simulink model "furuta_block_model_fixed_ppo_swingup"  (R2026b)
settings: Solver=ode14x  StopTime=25  FixedStep=driveElectrical.sampleTime
InitFcn:
  | validate_furuta_fixed_test(bdroot);
model workspace (MAT data in the model file):
  calibration = [73.65 -1 4058.5 1]
  controlPeriod = 0.01
  drive = [-1 1.5 1.5 inf]
  driveElectrical : object (value not decoded)
  failureReplayEnabled = 0
  failureReplaySlowdown = 10
  failureReplaySource = 'C:\Capstone1\matlab_furuta\results\ppo_rmd_candidate_tpa79dc374_f9fe_4d66_a12a_2e210f4a8415\ppo_start_-20_+20_armrate_20_current_1.5_time_10_armlimit_Inf.mat'
  failureReplayStartDeg = 20
  failureReplayState = [0 0.1 0.2 0.3 0.4 0.5 0.6 0.7 0.8 0.9 1 1.1 ... (205 elements, 41x5)]
  furutaPPOAgent : rl.agent.rlPPOAgent (value not decoded)
  furutaSACAgent : rl.agent.rlSACAgent (value not decoded)
  furutaToolboxMpc : object (value not decoded)
  initialState = [0; 3.14159265359; 0; 0]
  integrationStep = 0.002
  limits = [inf 3.3 15 20]
  lqrGain = [-1.90684760658 -25.0276005412 -1.03983138576 -2.50199272238]
  maxTorque = 3.15
  milVelocityLimits = [15 25]
  pidGains = [25.0276005412 5.00398544475 1.90684760658 2.07966277151 0.001]
  plantCoefficients = [0.05 0.00016078 0.00016134 0.00013805 0.016934 0.0001 1e-05 0.63]
  rlRewardLevel = 2
  rmd : object (value not decoded)
  rmdCommandDelaySamples = 1
  scenarioStimulus = [0  0  0  0; 20  0  0  0]
  swingLqrThresholds = [0.226892802759 0.2 0.523598775598]
  usePolicyCallback = 0
  useRmd = 1
  velocityFilterTau = 0.03
values from neighbouring files (symbols this model uses):
  C = [B A*B A^2*B A^3*B]    [build_furuta_rmd.m]
  N = 20    [build_furuta_rl.m]    (also in design_classical.m)
  s = load(matFile,'ds')    [analyze_pi_current_run.m]    (also in analyze_pi_speed_run.m; build_furuta_rl.m = sin(x(2));"; build_furuta_simulink.m = s(1); design_classical.m = furuta_scenarios)
  source = [step '/1']    [add_furuta_plant_blocks.m]    (also in build_furuta_pi.m = get_param(line,'SrcPortHandle'); build_furuta_pi_hardware.m = 'Drive interlocks/3'; compare_furuta_actuators.m = get_param([harness '/Requested torque'],'PortHandles'))
  Z = expm([A B; zeros(1,5)]*p.Ts)    [furuta_linearize.m]
symbols that are objects in the model workspace (value not decoded): driveElectrical, rmd
undefined symbols (not defined in the file or in its folder): lmpcF, lmpcH, poleGain, sgn, X, Y
libraries: sm_lib x36, raspberrypiCommlib x9, nesl_utility x8, fl_lib x7, rllib x2, mpclib x1, slpidlib x1, ee_lib x1
(part 3 of 4)

== system furuta_block_model_fixed_ppo_swingup/01 MIL - Controller and Plant/03 Controllers/PID ==
  mode : Inport
  x : Inport  Port=2
  Arm reference log : ToWorkspace  VariableName=swingPIDArmHome  SaveFormat=Timeseries  SampleTime=-1
  Capture arm reference : MATLAB Function  TreatAsAtomicUnit=on
  Capture thresholds : Constant  Value=swingLqrThresholds
  Control period : Constant  Value=controlPeriod
  Energy parameters : Constant  Value=plantCoefficients
  PID Controller : slpidlib/PID Controller  Controller=PID  Form=Parallel  TimeDomain=Continuous-time  UseExternalTs=off  SampleTime=-1  IntegratorMethod=Forward Euler  FilterMethod=Forward Euler  ControllerParametersSource=internal  P=1  I=1  UseKiTs=off  D=0  UseExternalDerivativeSource=off  N=100  UseFilter=on  TunerSelectOption=Transfer Function Based (PID Tuner App)  InitialConditionSource=internal  InitialConditionForIntegrator=0  InitialConditionForFilter=0  DifferentiatorICPrevScaledInput=0  ExternalReset=none  TrackingMode=off  Kt=1  LimitOutput=off  SatLimitsSource=internal  UpperSaturationLimit=inf  LowerSaturationLimit=-inf  LinearizeAsGain=on  AntiWindupMode=none  Kb=1  LimitIntegrator=off  UpperIntegratorSaturationLimit=inf  LowerIntegratorSaturationLimit=-inf  POutMin=[]  POutMax=[]  IOutMin=[]  IOutMax=[]  DOutMin=[]  DOutMax=[]  NOutMin=[]  NOutMax=[]  SumOutMin=[]  SumOutMax=[]  SaturationOutMin=[]  SaturationOutMax=[]  PParamMin=[]  PParamMax=[]  IParamMin=[]  IParamMax=[]  DParamMin=[]  DParamMax=[]  NParamMin=[]  NParamMax=[]  KbParamMin=[]  KbParamMax=[]  KtParamMin=[]  KtParamMax=[]  KbOutMin=[]  KbOutMax=[]  KtOutMin=[]  KtOutMax=[]  IntegratorOutMin=[]  IntegratorOutMax=[]  FilterOutMin=[]  FilterOutMax=[]  SumI1OutMin=[]  SumI1OutMax=[]  SumI2OutMin=[]  SumI2OutMax=[]  SumI3OutMin=[]  SumI3OutMax=[]  SumI4OutMin=[]  SumI4OutMax=[]  SumDOutMin=[]  SumDOutMax=[]  DifferentiatorOutMin=[]  DifferentiatorOutMax=[]  FilterDiffOutCoefMin=[]  FilterDiffOutCoefMax=[]  ReciprocalOutMin=[]  ReciprocalOutMax=[]  SumDenOutMin=[]  SumDenOutMax=[]  SumNumOutMin=[]  SumNumOutMax=[]  DivideOutMin=[]  DivideOutMax=[]  UdiffTsProdOutMin=[]  UdiffTsProdOutMax=[]  NTsProdOutMin=[]  NTsProdOutMax=[]  UintegralTsProdOutMin=[]  UintegralTsProdOutMax=[]  UngainTsProdOutMin=[]  UngainTsProdOutMax=[]  ClampingZeroOutDataTypeStr=Inherit: Inherit via back propagation  ClampingZeroOutMin=[]  ClampingZeroOutMax=[]  FilterDenConstantOutDataTypeStr=Inherit: Inherit via back propagation  FilterDenConstantOutMin=[]  FilterDenConstantOutMax=[]  PCopyOutDataTypeStr=Inherit: Inherit via back propagation  PCopyOutMin=[]  PCopyOutMax=[]  NCopyOutDataTypeStr=Inherit: Inherit via back propagation  NCopyOutMin=[]  NCopyOutMax=[]  IntegratorContinuousStateAttributes=''  IntegratorStateMustResolveToSignalObject=off  IntegratorRTWStateStorageClass=Auto  FilterContinuousStateAttributes=''  FilterStateMustResolveToSignalObject=off  FilterRTWStateStorageClass=Auto  ParallelPVariant=InternalParameters  IdealPVariant=Disabled  IVariant=InternalParameters  DVariant=InternalParameters  IntegratorVariant=Continuous  SatVariant=Disabled  AWVariant=Passthrough  PCopyVariant=Disabled  TRVariant=Disabled  FdbkBlocksVariant=Forward  IdealPFdbkVariant=Disabled  SatFdbkVariant=Disabled  DerivativeFilterVariant=ContFilter  NVariant=InternalParameters  NCopyVariant=Disabled  FilterICVariant=InternalICsFilter  IntegratorICVariant=InternalICs  ExternalResetVariant=Disabled  TRSumVariant=Passthrough  SumFdbkVariant=Disabled  SumVariant=Sum_PID  TsampFilterVariant=InternalTs  TsampNgainVariant=Passthrough  TsampIntegralVariant=Disabled_SignalSpec  ExternalSaturationOutDataTypeStr=Inherit: Same as second input  DerivativeSourceVariant=ErrorSignal  PreIntVariant=InternalPreInt
  PID active log : ToWorkspace  VariableName=swingPIDActive  SaveFormat=Timeseries  SampleTime=-1
  PID gains : Constant  Value=pidGains
  PID with anti windup : MATLAB Function  TreatAsAtomicUnit=on
  Swing-up to PID : MATLAB Function  TreatAsAtomicUnit=on
  u : Outport
  wires:
  PID gains/1 -> PID with anti windup/2(g)
  Control period/1 -> PID with anti windup/3(dt)
  x/1 -> Swing-up to PID/1(x), Capture arm reference/1(x)
  mode/1 -> Swing-up to PID/3(mode), Capture arm reference/2(mode)
  PID with anti windup/1(u) -> Swing-up to PID/2(balance)
  Capture thresholds/1 -> Swing-up to PID/4(thresholds), Capture arm reference/3(thresholds)
  Energy parameters/1 -> Swing-up to PID/5(p)
  Swing-up to PID/1(u) -> u/1
  Swing-up to PID/2(balancing) -> PID active log/1
  Capture arm reference/1(relative) -> PID with anti windup/1(x)
  Capture arm reference/2(gatedMode) -> PID with anti windup/4(mode)
  Capture arm reference/3(home) -> Arm reference log/1

== system furuta_block_model_fixed_ppo_swingup/01 MIL - Controller and Plant/03 Controllers/PPO ==
  Controller mode : Inport
  Measured state : Inport  Port=2
  Previous RL action : UnitDelay  SampleTime=controlPeriod
  RL Agent : rllib/RL Agent  Agent=furutaPPOAgent  ExternalActionAsInput=off  ProvideLastAction=off  ProvideCumRwd=off  TreatAsDirectFeedthrough=on  UseStrictObservationDataTypes=off
  RL action limit : Saturate  UpperLimit=1  LowerLimit=-1
  RL observation reward termination : MATLAB Function  TreatAsAtomicUnit=on
  Reward level : Constant  Value=rlRewardLevel
  Out1 : Outport
  wires:
  Controller mode/1 -> RL observation reward termination/1(x)
  RL observation reward termination/3(done) -> RL Agent/3
  RL Agent/1 -> RL action limit/1
  RL observation reward termination/2(reward) -> RL Agent/2
  Previous RL action/1 -> RL observation reward termination/2(lastAction)
  RL action limit/1 -> Out1/1, Previous RL action/1
  RL observation reward termination/1(obs) -> RL Agent/1
  Reward level/1 -> RL observation reward termination/3(level)
  Measured state/1 -> RL observation reward termination/4(mode)

== system furuta_block_model_fixed_ppo_swingup/01 MIL - Controller and Plant/03 Controllers/Pendulum and arm PD ==
  mode : Inport
  x : Inport  Port=2
  Control period : Constant  Value=controlPeriod
  Pendulum and arm PD : Gain  Gain=[.50 8.0 .29 .58]  Multiplication=Matrix(K*u) (u vector)
  u : Outport
  wires:
  Control period/1 -> ?
  mode/1 -> ?
  Pendulum and arm PD/1 -> u/1
  x/1 -> Pendulum and arm PD/1

== system furuta_block_model_fixed_ppo_swingup/01 MIL - Controller and Plant/03 Controllers/Pole placement ==
  mode : Inport
  x : Inport  Port=2
  Control period : Constant  Value=controlPeriod
  Pole placement : Gain  Gain=-poleGain  Multiplication=Matrix(K*u) (u vector)
  u : Outport
  wires:
  Control period/1 -> ?
  mode/1 -> ?
  Pole placement/1 -> u/1
  x/1 -> Pole placement/1

== system furuta_block_model_fixed_ppo_swingup/01 MIL - Controller and Plant/03 Controllers/SAC ==
  x : Inport
  mode : Inport  Port=2
  Previous RL action : UnitDelay  SampleTime=controlPeriod
  RL Agent : rllib/RL Agent  Agent=furutaSACAgent  ExternalActionAsInput=off  ProvideLastAction=off  ProvideCumRwd=off  TreatAsDirectFeedthrough=on  UseStrictObservationDataTypes=off
  RL action limit : Saturate  UpperLimit=1  LowerLimit=-1
  RL observation reward termination : MATLAB Function  TreatAsAtomicUnit=on
  Reward level : Constant  Value=rlRewardLevel
  Out1 : Outport
  wires:
  x/1 -> RL observation reward termination/1(x)
  RL observation reward termination/3(done) -> RL Agent/3
  RL Agent/1 -> RL action limit/1
  RL observation reward termination/2(reward) -> RL Agent/2
  Previous RL action/1 -> RL observation reward termination/2(lastAction)
  RL action limit/1 -> Out1/1, Previous RL action/1
  RL observation reward termination/1(obs) -> RL Agent/1
  Reward level/1 -> RL observation reward termination/3(level)
  mode/1 -> RL observation reward termination/4(mode)

== system furuta_block_model_fixed_ppo_swingup/01 MIL - Controller and Plant/04 Actuator/RMD X6 P20 60 E ==
  Output shaft speed : Inport
  Requested torque : Inport  Port=2
  01 RMD Driver : Subsystem
  02 RMD Motor : Subsystem
  Output torque : Outport
  wires:
  Requested torque/1 -> 01 RMD Driver/2(Requested torque)
  Output shaft speed/1 -> 02 RMD Motor/1(Output shaft speed)
  02 RMD Motor/1(output) -> 01 RMD Driver/1(output)
  02 RMD Motor/2(input0) -> 01 RMD Driver/3(input0)
  02 RMD Motor/3(Output torque) -> Output torque/1
  connections:
  01 RMD Driver/RConn1 -- 02 RMD Motor/LConn1
  02 RMD Motor/RConn1 -- 01 RMD Driver/LConn1

== system furuta_block_model_fixed_ppo_swingup/01 MIL - Controller and Plant/05 Furuta plant/RK4 Furuta plant ==
  state : Inport
  total torque : Inport  Port=2
  Substep 1 : Subsystem
  Substep 2 : Subsystem
  Substep 3 : Subsystem
  Substep 4 : Subsystem
  Substep 5 : Subsystem
  next state : Outport
  wires:
  state/1 -> Substep 1/1(x)
  total torque/1 -> Substep 4/2(tau), Substep 5/2(tau), Substep 3/2(tau), Substep 2/2(tau), Substep 1/2(tau)
  Substep 1/1(x next) -> Substep 2/1(x)
  Substep 2/1(x next) -> Substep 3/1(x)
  Substep 3/1(x next) -> Substep 4/1(x)
  Substep 4/1(x next) -> Substep 5/1(x)
  Substep 5/1(x next) -> next state/1

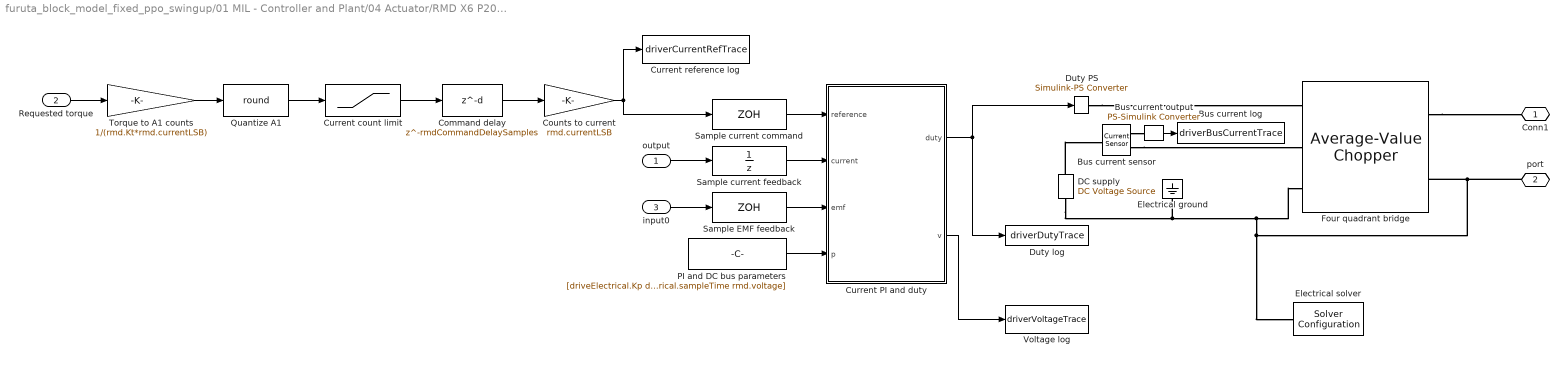
== system furuta_block_model_fixed_ppo_swingup/01 MIL - Controller and Plant/04 Actuator/RMD X6 P20 60 E/01 RMD Driver ==
  output : Inport
  Requested torque : Inport  Port=2
  input0 : Inport  Port=3
  Bus current log : ToWorkspace  VariableName=driverBusCurrentTrace  SaveFormat=Timeseries  SampleTime=-1
  Bus current output : nesl_utility/PS-Simulink Converter  PhysicalDomain=network_engine_domain  SubClassName=ps_output  LeftPortType=input  RightPortType=output  PseudoPeriodic=off  Frequencies=[]  VectorFormat=inherit  Unit=A  AffineConversion=off
  Bus current sensor : fl_lib/Electrical/Electrical Sensors/Current Sensor
  Command delay : Delay  DelayLength=rmdCommandDelaySamples  SampleTime=controlPeriod
  Counts to current : Gain  Gain=rmd.currentLSB
  Current PI and duty : MATLAB Function  TreatAsAtomicUnit=on
  Current count limit : Saturate  UpperLimit=floor(min([maxTorque/rmd.Kt rmd.ratedTorque/rmd.Kt rmd.ratedCurrent])/rmd.currentLSB)  LowerLimit=-(floor(min([maxTorque/rmd.Kt rmd.ratedTorque/rmd.Kt rmd.ratedCurrent])/rmd.currentLSB))
  Current reference log : ToWorkspace  VariableName=driverCurrentRefTrace  SaveFormat=Timeseries  SampleTime=-1
  DC supply : fl_lib/Electrical/Electrical Sources/DC Voltage Source  v0=rmd.voltage V
  Duty PS : nesl_utility/Simulink-PS Converter  PhysicalDomain=network_engine_domain  SubClassName=ps_input  LeftPortType=input  RightPortType=output  PseudoPeriodic=off  Frequencies=[]  NoiseDistribution=none  NoiseParameters=[]  Unit=1  AffineConversion=off  FilteringAndDerivatives=zero  SimscapeFilterOrder=1  InputFilterTimeConstant=0.001  UdotUserProvided=0
  Duty log : ToWorkspace  VariableName=driverDutyTrace  SaveFormat=Timeseries  SampleTime=-1
  Electrical ground : fl_lib/Electrical/Electrical Elements/Electrical Reference
  Electrical solver : nesl_utility/Solver Configuration  PhysicalDomain=network_engine_domain  SubClassName=solver  LeftPortType=input  RightPortType=generic  Tones=[]  Harmonics=[]  SimulateNoise=off  Profile=off  UseLocalSampling=off  EnableSwitchedLinearOptims=on  FrequencyDomain=off  UseCCode=off  RelTol=0.001  AbsTol=0.001  MinStep=1e-09  ToWorkspace=off  RevertToSquareIcSolve=off  NumHomotopyIterations=100  PhasorMode=off  PhasorModeNumHarmonics=1  ConsistencySolver=NEWTON_XTOL_AFTER_FTOL  CanonicalOrdering=CANONICAL  OptimizeIntermediates=OPTIMIZED  MulticoreSolverChoice=BACKWARD_EULER  IndexReductionMethod=DerivativeReplacement  DoDC=off  ResidualTolerance=1e-09  ConsistencyTolSource=GLOBAL  ConsistencyAbsTol=0.001  ConsistencyRelTol=0.001  ConsistencyTolFactor=0.001  UseLocalSolver=off  LocalSolverChoice=NE_BACKWARD_EULER_ADVANCER  ResolveIndetEquations=on  FunctionEvalNumThread=1  LocalSolverSampleTime=0.001  DoFixedCost=off  MaxNonlinIter=3  MaxModeIter=2  ComputeImpulses=off  ImpulseIterations=2  LinearAlgebra=auto  LinearAlgebraNumThread=0  EquationFormulation=NE_TIME_EF  DelaysMemoryBudget=1024  AutomaticFiltering=on  FilteringTimeConstant=0.001  PartitionStorageMethod=AS_NEEDED  PartitionMemoryBudget=1024  PartitionMethod=BALANCED  MultibodyUseLocalSolver=off  MultibodyLocalSolverChoice=ODE1  MultibodyLocalSolverSampleTime=0.001
  Four quadrant bridge : ee_lib/Semiconductors & Converters/Converters/Average-Value Chopper  chopper_type=ee.enum.converters.averageChopperType.classE  efficiency_option=ee.enum.converters.efficiencyOption.constant  efficiency_fixed=100  i_vec=[0, 2, 5] A  efficiency_vec=[90, 95, 98]
  PI and DC bus parameters : Constant  Value=[driveElectrical.Kp driveElectrical.Ki driveElectrical.sampleTime rmd.voltage]
  Quantize A1 : Rounding  Operator=round
  Sample EMF feedback : ZeroOrderHold  SampleTime=driveElectrical.sampleTime
  Sample current command : ZeroOrderHold  SampleTime=driveElectrical.sampleTime
  Sample current feedback : UnitDelay  SampleTime=driveElectrical.sampleTime
  Torque to A1 counts : Gain  Gain=1/(rmd.Kt*rmd.currentLSB)
  Voltage log : ToWorkspace  VariableName=driverVoltageTrace  SaveFormat=Timeseries  SampleTime=-1
  Conn1 : PMIOPort  Side=Right
  port : PMIOPort  Port=2  Side=Left
  wires:
  Torque to A1 counts/1 -> Quantize A1/1
  Command delay/1 -> Counts to current/1
  Bus current output/1 -> Bus current log/1
  Sample current command/1 -> Current PI and duty/1(reference)
  Counts to current/1 -> Current reference log/1, Sample current command/1
  Current count limit/1 -> Command delay/1
  Quantize A1/1 -> Current count limit/1
  Current PI and duty/1(duty) -> Duty PS/1, Duty log/1
  Sample current feedback/1 -> Current PI and duty/2(current)
  input0/1 -> Sample EMF feedback/1
  Current PI and duty/2(v) -> Voltage log/1
  Sample EMF feedback/1 -> Current PI and duty/3(emf)
  PI and DC bus parameters/1 -> Current PI and duty/4(p)
  output/1 -> Sample current feedback/1
  Requested torque/1 -> Torque to A1 counts/1
  connections:
  Bus current sensor/RConn1 -- Bus current output/LConn1
  port/RConn1 -- Four quadrant bridge/RConn2 -- Electrical solver/RConn1 -- Four quadrant bridge/LConn3 -- DC supply/RConn1 -- Electrical ground/LConn1
  Duty PS/RConn1 -- Four quadrant bridge/LConn1
  DC supply/LConn1 -- Bus current sensor/LConn1
  Bus current sensor/RConn2 -- Four quadrant bridge/LConn2
  Four quadrant bridge/RConn1 -- Conn1/RConn1

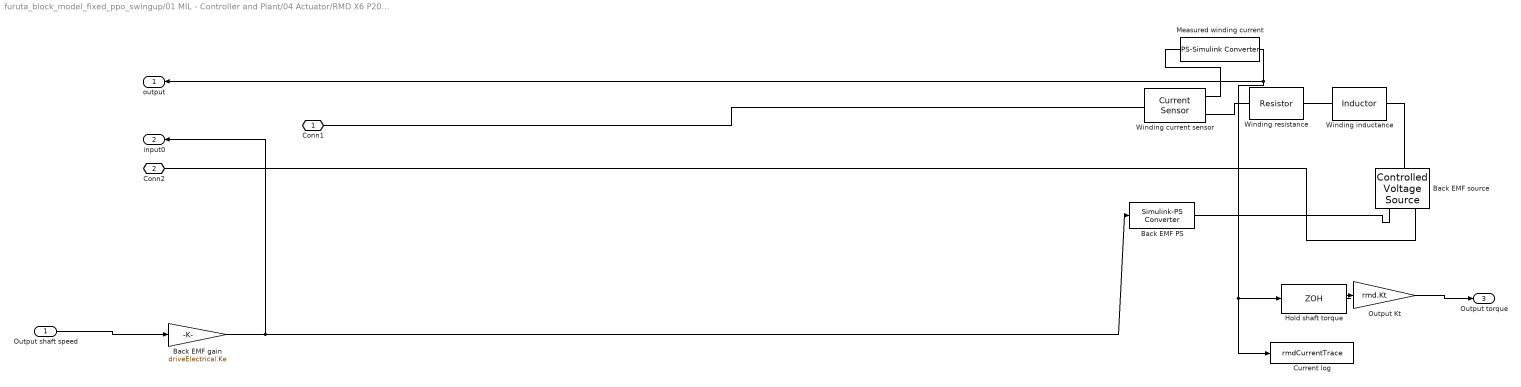
== system furuta_block_model_fixed_ppo_swingup/01 MIL - Controller and Plant/04 Actuator/RMD X6 P20 60 E/02 RMD Motor ==
  Output shaft speed : Inport
  Back EMF PS : nesl_utility/Simulink-PS Converter  PhysicalDomain=network_engine_domain  SubClassName=ps_input  LeftPortType=input  RightPortType=output  PseudoPeriodic=off  Frequencies=[]  NoiseDistribution=none  NoiseParameters=[]  Unit=V  AffineConversion=off  FilteringAndDerivatives=zero  SimscapeFilterOrder=1  InputFilterTimeConstant=0.001  UdotUserProvided=0
  Back EMF gain : Gain  Gain=driveElectrical.Ke
  Back EMF source : fl_lib/Electrical/Electrical Sources/Controlled Voltage Source
  Current log : ToWorkspace  VariableName=rmdCurrentTrace  SampleTime=-1
  Hold shaft torque : ZeroOrderHold  SampleTime=controlPeriod
  Measured winding current : nesl_utility/PS-Simulink Converter  PhysicalDomain=network_engine_domain  SubClassName=ps_output  LeftPortType=input  RightPortType=output  PseudoPeriodic=off  Frequencies=[]  VectorFormat=inherit  Unit=A  AffineConversion=off
  Output Kt : Gain  Gain=rmd.Kt
  Winding current sensor : fl_lib/Electrical/Electrical Sensors/Current Sensor
  Winding inductance : fl_lib/Electrical/Electrical Elements/Inductor  l=driveElectrical.L H  r=0 Ohm  g=0 1/Ohm  i_specify=off  i_priority=None  i=0 A  i_nominal_specify=off  i_nominal_value=1  i_nominal_unit=A  v_specify=off  v_priority=None  v=0 V  v_nominal_specify=off  v_nominal_value=1  v_nominal_unit=V  i_L_specify=off  i_L_priority=High  i_L=0 A  i_L_nominal_specify=off  i_L_nominal_value=1  i_L_nominal_unit=A
  Winding resistance : fl_lib/Electrical/Electrical Elements/Resistor  R=driveElectrical.R Ohm  i_specify=off  i_priority=None  i=0 A  i_nominal_specify=off  i_nominal_value=1  i_nominal_unit=A  v_specify=off  v_priority=None  v=0 V  v_nominal_specify=off  v_nominal_value=1  v_nominal_unit=V
  Conn1 : PMIOPort  Side=Left
  Conn2 : PMIOPort  Port=2  Side=Right
  output : Outport
  input0 : Outport  Port=2
  Output torque : Outport  Port=3
  wires:
  Measured winding current/1 -> output/1, Hold shaft torque/1, Current log/1
  Output Kt/1 -> Output torque/1
  Hold shaft torque/1 -> Output Kt/1
  Back EMF gain/1 -> Back EMF PS/1, input0/1
  Output shaft speed/1 -> Back EMF gain/1
  connections:
  Back EMF PS/RConn1 -- Back EMF source/RConn1
  Winding current sensor/RConn1 -- Measured winding current/LConn1
  Winding resistance/RConn1 -- Winding inductance/LConn1
  Winding inductance/RConn1 -- Back EMF source/LConn1
  Winding current sensor/RConn2 -- Winding resistance/LConn1
  Conn1/RConn1 -- Winding current sensor/LConn1
  Back EMF source/RConn2 -- Conn2/RConn1

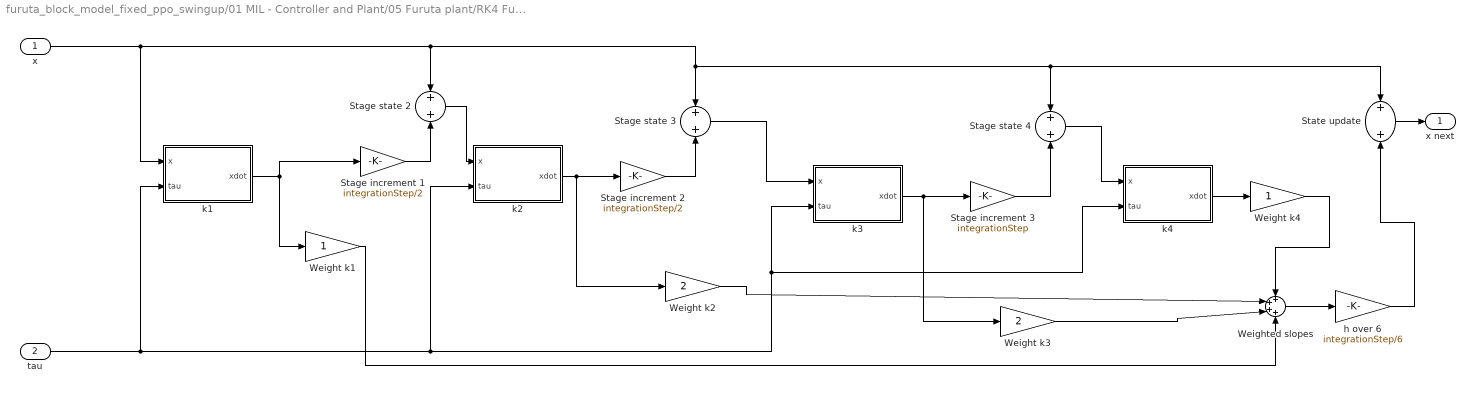
== system furuta_block_model_fixed_ppo_swingup/01 MIL - Controller and Plant/05 Furuta plant/RK4 Furuta plant/Substep 1 ==
  x : Inport
  tau : Inport  Port=2
  Stage increment 1 : Gain  Gain=integrationStep/2
  Stage increment 2 : Gain  Gain=integrationStep/2
  Stage increment 3 : Gain  Gain=integrationStep
  Stage state 2 : Sum
  Stage state 3 : Sum
  Stage state 4 : Sum
  State update : Sum
  Weight k1 : Gain
  Weight k2 : Gain  Gain=2
  Weight k3 : Gain  Gain=2
  Weight k4 : Gain
  Weighted slopes : Sum  Inputs=++++
  h over 6 : Gain  Gain=integrationStep/6
  k1 : Subsystem
  k2 : Subsystem
  k3 : Subsystem
  k4 : Subsystem
  x next : Outport
  wires:
  x/1 -> Stage state 3/1, Stage state 4/1, State update/1, Stage state 2/1, k1/1(x)
  tau/1 -> k4/2(tau), k3/2(tau), k2/2(tau), k1/2(tau)
  k1/1(xdot) -> Stage increment 1/1, Weight k1/1
  Stage increment 1/1 -> Stage state 2/2
  Stage state 2/1 -> k2/1(x)
  k2/1(xdot) -> Stage increment 2/1, Weight k2/1
  Stage increment 2/1 -> Stage state 3/2
  Stage state 3/1 -> k3/1(x)
  k3/1(xdot) -> Weight k3/1, Stage increment 3/1
  Stage increment 3/1 -> Stage state 4/2
  Stage state 4/1 -> k4/1(x)
  k4/1(xdot) -> Weight k4/1
  Weight k1/1 -> Weighted slopes/4
  Weight k2/1 -> Weighted slopes/2
  Weight k3/1 -> Weighted slopes/3
  Weight k4/1 -> Weighted slopes/1
  Weighted slopes/1 -> h over 6/1
  h over 6/1 -> State update/2
  State update/1 -> x next/1

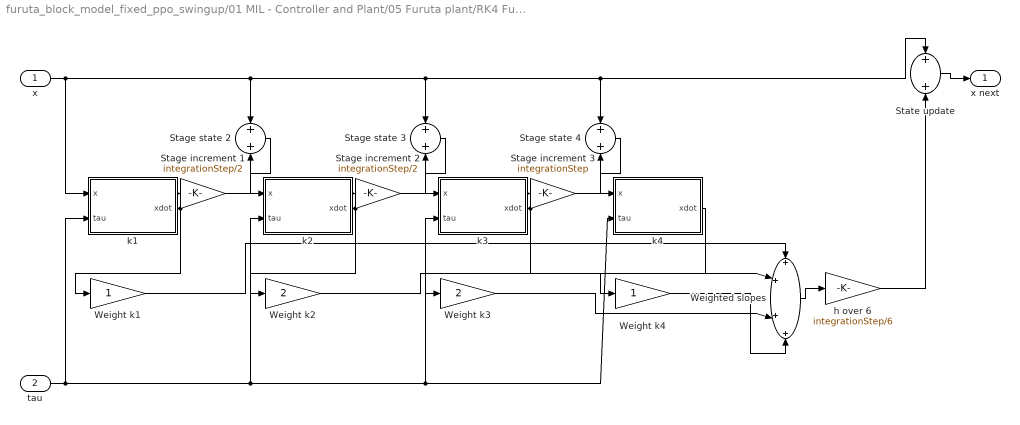
== system furuta_block_model_fixed_ppo_swingup/01 MIL - Controller and Plant/05 Furuta plant/RK4 Furuta plant/Substep 2 ==
  x : Inport
  tau : Inport  Port=2
  Stage increment 1 : Gain  Gain=integrationStep/2
  Stage increment 2 : Gain  Gain=integrationStep/2
  Stage increment 3 : Gain  Gain=integrationStep
  Stage state 2 : Sum
  Stage state 3 : Sum
  Stage state 4 : Sum
  State update : Sum
  Weight k1 : Gain
  Weight k2 : Gain  Gain=2
  Weight k3 : Gain  Gain=2
  Weight k4 : Gain
  Weighted slopes : Sum  Inputs=++++
  h over 6 : Gain  Gain=integrationStep/6
  k1 : Subsystem
  k2 : Subsystem
  k3 : Subsystem
  k4 : Subsystem
  x next : Outport
  wires:
  State update/1 -> x next/1
  h over 6/1 -> State update/2
  Weighted slopes/1 -> h over 6/1
  Weight k4/1 -> Weighted slopes/4
  Weight k3/1 -> Weighted slopes/3
  Weight k2/1 -> Weighted slopes/2
  Weight k1/1 -> Weighted slopes/1
  k4/1(xdot) -> Weight k4/1
  Stage state 4/1 -> k4/1(x)
  Stage increment 3/1 -> Stage state 4/2
  k3/1(xdot) -> Weight k3/1, Stage increment 3/1
  Stage state 3/1 -> k3/1(x)
  Stage increment 2/1 -> Stage state 3/2
  k2/1(xdot) -> Weight k2/1, Stage increment 2/1
  Stage state 2/1 -> k2/1(x)
  Stage increment 1/1 -> Stage state 2/2
  k1/1(xdot) -> Weight k1/1, Stage increment 1/1
  tau/1 -> k4/2(tau), k3/2(tau), k2/2(tau), k1/2(tau)
  x/1 -> State update/1, Stage state 4/1, Stage state 3/1, Stage state 2/1, k1/1(x)

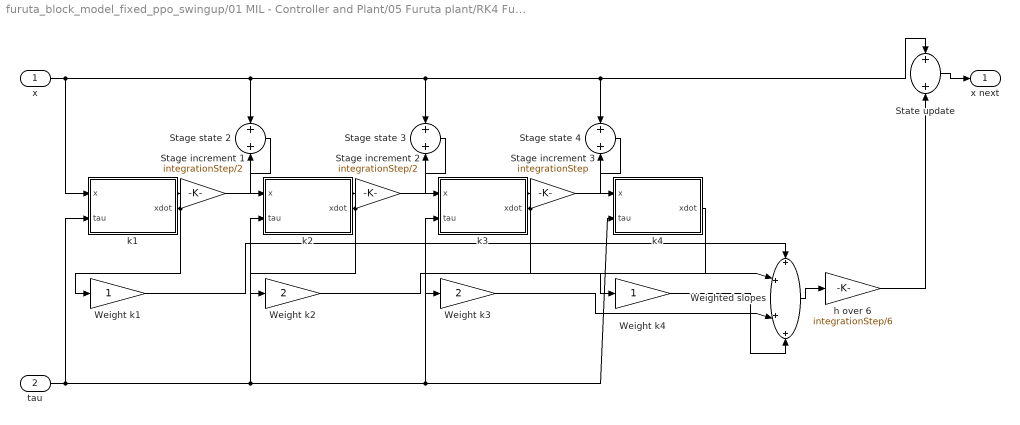
== system furuta_block_model_fixed_ppo_swingup/01 MIL - Controller and Plant/05 Furuta plant/RK4 Furuta plant/Substep 3 ==
  x : Inport
  tau : Inport  Port=2
  Stage increment 1 : Gain  Gain=integrationStep/2
  Stage increment 2 : Gain  Gain=integrationStep/2
  Stage increment 3 : Gain  Gain=integrationStep
  Stage state 2 : Sum
  Stage state 3 : Sum
  Stage state 4 : Sum
  State update : Sum
  Weight k1 : Gain
  Weight k2 : Gain  Gain=2
  Weight k3 : Gain  Gain=2
  Weight k4 : Gain
  Weighted slopes : Sum  Inputs=++++
  h over 6 : Gain  Gain=integrationStep/6
  k1 : Subsystem
  k2 : Subsystem
  k3 : Subsystem
  k4 : Subsystem
  x next : Outport
  wires:
  State update/1 -> x next/1
  h over 6/1 -> State update/2
  Weighted slopes/1 -> h over 6/1
  Weight k4/1 -> Weighted slopes/4
  Weight k3/1 -> Weighted slopes/3
  Weight k2/1 -> Weighted slopes/2
  Weight k1/1 -> Weighted slopes/1
  k4/1(xdot) -> Weight k4/1
  Stage state 4/1 -> k4/1(x)
  Stage increment 3/1 -> Stage state 4/2
  k3/1(xdot) -> Weight k3/1, Stage increment 3/1
  Stage state 3/1 -> k3/1(x)
  Stage increment 2/1 -> Stage state 3/2
  k2/1(xdot) -> Weight k2/1, Stage increment 2/1
  Stage state 2/1 -> k2/1(x)
  Stage increment 1/1 -> Stage state 2/2
  k1/1(xdot) -> Weight k1/1, Stage increment 1/1
  tau/1 -> k4/2(tau), k3/2(tau), k2/2(tau), k1/2(tau)
  x/1 -> State update/1, Stage state 4/1, Stage state 3/1, Stage state 2/1, k1/1(x)

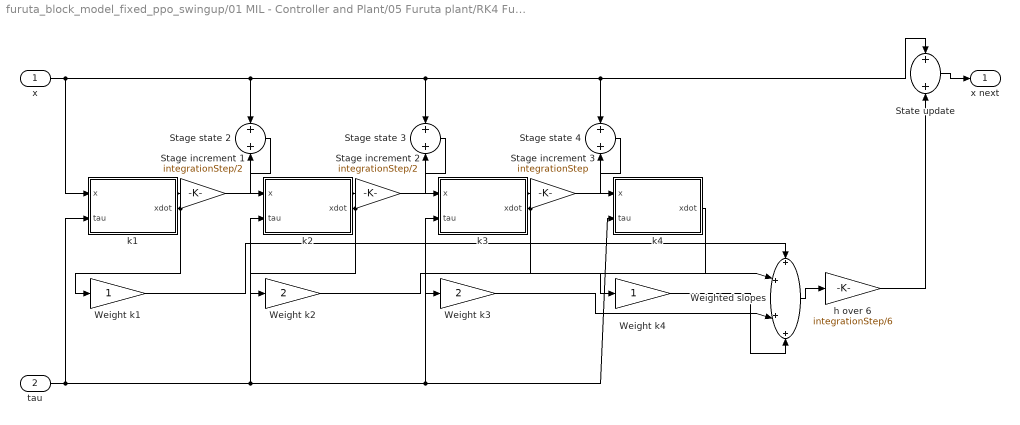
== system furuta_block_model_fixed_ppo_swingup/01 MIL - Controller and Plant/05 Furuta plant/RK4 Furuta plant/Substep 4 ==
  x : Inport
  tau : Inport  Port=2
  Stage increment 1 : Gain  Gain=integrationStep/2
  Stage increment 2 : Gain  Gain=integrationStep/2
  Stage increment 3 : Gain  Gain=integrationStep
  Stage state 2 : Sum
  Stage state 3 : Sum
  Stage state 4 : Sum
  State update : Sum
  Weight k1 : Gain
  Weight k2 : Gain  Gain=2
  Weight k3 : Gain  Gain=2
  Weight k4 : Gain
  Weighted slopes : Sum  Inputs=++++
  h over 6 : Gain  Gain=integrationStep/6
  k1 : Subsystem
  k2 : Subsystem
  k3 : Subsystem
  k4 : Subsystem
  x next : Outport
  wires:
  State update/1 -> x next/1
  h over 6/1 -> State update/2
  Weighted slopes/1 -> h over 6/1
  Weight k4/1 -> Weighted slopes/4
  Weight k3/1 -> Weighted slopes/3
  Weight k2/1 -> Weighted slopes/2
  Weight k1/1 -> Weighted slopes/1
  k4/1(xdot) -> Weight k4/1
  Stage state 4/1 -> k4/1(x)
  Stage increment 3/1 -> Stage state 4/2
  k3/1(xdot) -> Weight k3/1, Stage increment 3/1
  Stage state 3/1 -> k3/1(x)
  Stage increment 2/1 -> Stage state 3/2
  k2/1(xdot) -> Weight k2/1, Stage increment 2/1
  Stage state 2/1 -> k2/1(x)
  Stage increment 1/1 -> Stage state 2/2
  k1/1(xdot) -> Weight k1/1, Stage increment 1/1
  tau/1 -> k4/2(tau), k3/2(tau), k2/2(tau), k1/2(tau)
  x/1 -> State update/1, Stage state 4/1, Stage state 3/1, Stage state 2/1, k1/1(x)

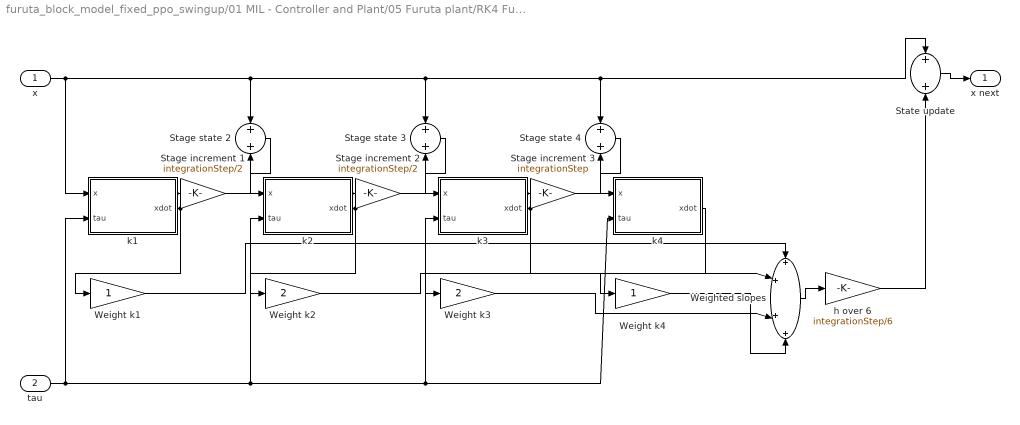
== system furuta_block_model_fixed_ppo_swingup/01 MIL - Controller and Plant/05 Furuta plant/RK4 Furuta plant/Substep 5 ==
  x : Inport
  tau : Inport  Port=2
  Stage increment 1 : Gain  Gain=integrationStep/2
  Stage increment 2 : Gain  Gain=integrationStep/2
  Stage increment 3 : Gain  Gain=integrationStep
  Stage state 2 : Sum
  Stage state 3 : Sum
  Stage state 4 : Sum
  State update : Sum
  Weight k1 : Gain
  Weight k2 : Gain  Gain=2
  Weight k3 : Gain  Gain=2
  Weight k4 : Gain
  Weighted slopes : Sum  Inputs=++++
  h over 6 : Gain  Gain=integrationStep/6
  k1 : Subsystem
  k2 : Subsystem
  k3 : Subsystem
  k4 : Subsystem
  x next : Outport
  wires:
  State update/1 -> x next/1
  h over 6/1 -> State update/2
  Weighted slopes/1 -> h over 6/1
  Weight k4/1 -> Weighted slopes/4
  Weight k3/1 -> Weighted slopes/3
  Weight k2/1 -> Weighted slopes/2
  Weight k1/1 -> Weighted slopes/1
  k4/1(xdot) -> Weight k4/1
  Stage state 4/1 -> k4/1(x)
  Stage increment 3/1 -> Stage state 4/2
  k3/1(xdot) -> Weight k3/1, Stage increment 3/1
  Stage state 3/1 -> k3/1(x)
  Stage increment 2/1 -> Stage state 3/2
  k2/1(xdot) -> Weight k2/1, Stage increment 2/1
  Stage state 2/1 -> k2/1(x)
  Stage increment 1/1 -> Stage state 2/2
  k1/1(xdot) -> Weight k1/1, Stage increment 1/1
  tau/1 -> k4/2(tau), k3/2(tau), k2/2(tau), k1/2(tau)
  x/1 -> State update/1, Stage state 4/1, Stage state 3/1, Stage state 2/1, k1/1(x)

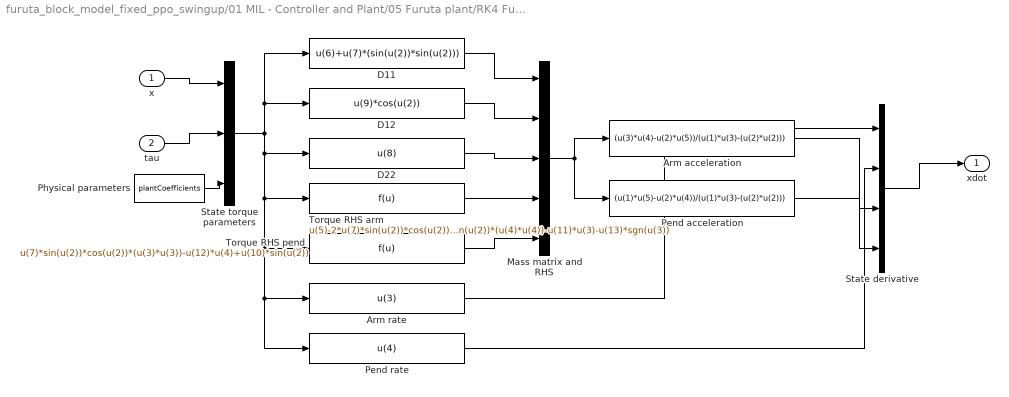
== system furuta_block_model_fixed_ppo_swingup/01 MIL - Controller and Plant/05 Furuta plant/RK4 Furuta plant/Substep 1/k1 ==
  x : Inport
  tau : Inport  Port=2
  Arm acceleration : Fcn  Expr=(u(3)*u(4)-u(2)*u(5))/(u(1)*u(3)-(u(2)*u(2)))
  Arm rate : Fcn  Expr=u(3)
  D11 : Fcn  Expr=u(6)+u(7)*(sin(u(2))*sin(u(2)))
  D12 : Fcn  Expr=u(9)*cos(u(2))
  D22 : Fcn  Expr=u(8)
  Mass matrix and RHS : Mux  Inputs=5
  Pend acceleration : Fcn  Expr=(u(1)*u(5)-u(2)*u(4))/(u(1)*u(3)-(u(2)*u(2)))
  Pend rate : Fcn  Expr=u(4)
  Physical parameters : Constant  Value=plantCoefficients
  State derivative : Mux
  State torque parameters : Mux  Inputs=3
  Torque RHS arm : Fcn  Expr=u(5)-2*u(7)*sin(u(2))*cos(u(2))*u(3)*u(4)+u(9)*sin(u(2))*(u(4)*u(4))-u(11)*u(3)-u(13)*sgn(u(3))
  Torque RHS pend : Fcn  Expr=u(7)*sin(u(2))*cos(u(2))*(u(3)*u(3))-u(12)*u(4)+u(10)*sin(u(2))
  xdot : Outport
  wires:
  x/1 -> State torque parameters/1
  tau/1 -> State torque parameters/2
  Physical parameters/1 -> State torque parameters/3
  State torque parameters/1 -> Arm rate/1, Pend rate/1, Torque RHS pend/1, Torque RHS arm/1, D22/1, D11/1, D12/1
  D11/1 -> Mass matrix and RHS/1
  D12/1 -> Mass matrix and RHS/2
  D22/1 -> Mass matrix and RHS/3
  Torque RHS arm/1 -> Mass matrix and RHS/4
  Torque RHS pend/1 -> Mass matrix and RHS/5
  Arm rate/1 -> State derivative/1
  Pend rate/1 -> State derivative/2
  Mass matrix and RHS/1 -> Arm acceleration/1, Pend acceleration/1
  Arm acceleration/1 -> State derivative/3
  Pend acceleration/1 -> State derivative/4
  State derivative/1 -> xdot/1

== system furuta_block_model_fixed_ppo_swingup/01 MIL - Controller and Plant/05 Furuta plant/RK4 Furuta plant/Substep 1/k2 ==
  x : Inport
  tau : Inport  Port=2
  Arm acceleration : Fcn  Expr=(u(3)*u(4)-u(2)*u(5))/(u(1)*u(3)-(u(2)*u(2)))
  Arm rate : Fcn  Expr=u(3)
  D11 : Fcn  Expr=u(6)+u(7)*(sin(u(2))*sin(u(2)))
  D12 : Fcn  Expr=u(9)*cos(u(2))
  D22 : Fcn  Expr=u(8)
  Mass matrix and RHS : Mux  Inputs=5
  Pend acceleration : Fcn  Expr=(u(1)*u(5)-u(2)*u(4))/(u(1)*u(3)-(u(2)*u(2)))
  Pend rate : Fcn  Expr=u(4)
  Physical parameters : Constant  Value=plantCoefficients
  State derivative : Mux
  State torque parameters : Mux  Inputs=3
  Torque RHS arm : Fcn  Expr=u(5)-2*u(7)*sin(u(2))*cos(u(2))*u(3)*u(4)+u(9)*sin(u(2))*(u(4)*u(4))-u(11)*u(3)-u(13)*sgn(u(3))
  Torque RHS pend : Fcn  Expr=u(7)*sin(u(2))*cos(u(2))*(u(3)*u(3))-u(12)*u(4)+u(10)*sin(u(2))
  xdot : Outport
  wires:
  State derivative/1 -> xdot/1
  Pend acceleration/1 -> State derivative/4
  Arm acceleration/1 -> State derivative/3
  Mass matrix and RHS/1 -> Pend acceleration/1, Arm acceleration/1
  Pend rate/1 -> State derivative/2
  Arm rate/1 -> State derivative/1
  Torque RHS pend/1 -> Mass matrix and RHS/5
  Torque RHS arm/1 -> Mass matrix and RHS/4
  D22/1 -> Mass matrix and RHS/3
  D12/1 -> Mass matrix and RHS/2
  D11/1 -> Mass matrix and RHS/1
  State torque parameters/1 -> Pend rate/1, Arm rate/1, Torque RHS pend/1, Torque RHS arm/1, D22/1, D12/1, D11/1
  Physical parameters/1 -> State torque parameters/3
  tau/1 -> State torque parameters/2
  x/1 -> State torque parameters/1

== system furuta_block_model_fixed_ppo_swingup/01 MIL - Controller and Plant/05 Furuta plant/RK4 Furuta plant/Substep 1/k3 ==
  x : Inport
  tau : Inport  Port=2
  Arm acceleration : Fcn  Expr=(u(3)*u(4)-u(2)*u(5))/(u(1)*u(3)-(u(2)*u(2)))
  Arm rate : Fcn  Expr=u(3)
  D11 : Fcn  Expr=u(6)+u(7)*(sin(u(2))*sin(u(2)))
  D12 : Fcn  Expr=u(9)*cos(u(2))
  D22 : Fcn  Expr=u(8)
  Mass matrix and RHS : Mux  Inputs=5
  Pend acceleration : Fcn  Expr=(u(1)*u(5)-u(2)*u(4))/(u(1)*u(3)-(u(2)*u(2)))
  Pend rate : Fcn  Expr=u(4)
  Physical parameters : Constant  Value=plantCoefficients
  State derivative : Mux
  State torque parameters : Mux  Inputs=3
  Torque RHS arm : Fcn  Expr=u(5)-2*u(7)*sin(u(2))*cos(u(2))*u(3)*u(4)+u(9)*sin(u(2))*(u(4)*u(4))-u(11)*u(3)-u(13)*sgn(u(3))
  Torque RHS pend : Fcn  Expr=u(7)*sin(u(2))*cos(u(2))*(u(3)*u(3))-u(12)*u(4)+u(10)*sin(u(2))
  xdot : Outport
  wires:
  State derivative/1 -> xdot/1
  Pend acceleration/1 -> State derivative/4
  Arm acceleration/1 -> State derivative/3
  Mass matrix and RHS/1 -> Pend acceleration/1, Arm acceleration/1
  Pend rate/1 -> State derivative/2
  Arm rate/1 -> State derivative/1
  Torque RHS pend/1 -> Mass matrix and RHS/5
  Torque RHS arm/1 -> Mass matrix and RHS/4
  D22/1 -> Mass matrix and RHS/3
  D12/1 -> Mass matrix and RHS/2
  D11/1 -> Mass matrix and RHS/1
  State torque parameters/1 -> Pend rate/1, Arm rate/1, Torque RHS pend/1, Torque RHS arm/1, D22/1, D12/1, D11/1
  Physical parameters/1 -> State torque parameters/3
  tau/1 -> State torque parameters/2
  x/1 -> State torque parameters/1

== system furuta_block_model_fixed_ppo_swingup/01 MIL - Controller and Plant/05 Furuta plant/RK4 Furuta plant/Substep 1/k4 ==
  x : Inport
  tau : Inport  Port=2
  Arm acceleration : Fcn  Expr=(u(3)*u(4)-u(2)*u(5))/(u(1)*u(3)-(u(2)*u(2)))
  Arm rate : Fcn  Expr=u(3)
  D11 : Fcn  Expr=u(6)+u(7)*(sin(u(2))*sin(u(2)))
  D12 : Fcn  Expr=u(9)*cos(u(2))
  D22 : Fcn  Expr=u(8)
  Mass matrix and RHS : Mux  Inputs=5
  Pend acceleration : Fcn  Expr=(u(1)*u(5)-u(2)*u(4))/(u(1)*u(3)-(u(2)*u(2)))
  Pend rate : Fcn  Expr=u(4)
  Physical parameters : Constant  Value=plantCoefficients
  State derivative : Mux
  State torque parameters : Mux  Inputs=3
  Torque RHS arm : Fcn  Expr=u(5)-2*u(7)*sin(u(2))*cos(u(2))*u(3)*u(4)+u(9)*sin(u(2))*(u(4)*u(4))-u(11)*u(3)-u(13)*sgn(u(3))
  Torque RHS pend : Fcn  Expr=u(7)*sin(u(2))*cos(u(2))*(u(3)*u(3))-u(12)*u(4)+u(10)*sin(u(2))
  xdot : Outport
  wires:
  State derivative/1 -> xdot/1
  Pend acceleration/1 -> State derivative/4
  Arm acceleration/1 -> State derivative/3
  Mass matrix and RHS/1 -> Pend acceleration/1, Arm acceleration/1
  Pend rate/1 -> State derivative/2
  Arm rate/1 -> State derivative/1
  Torque RHS pend/1 -> Mass matrix and RHS/5
  Torque RHS arm/1 -> Mass matrix and RHS/4
  D22/1 -> Mass matrix and RHS/3
  D12/1 -> Mass matrix and RHS/2
  D11/1 -> Mass matrix and RHS/1
  State torque parameters/1 -> Pend rate/1, Arm rate/1, Torque RHS pend/1, Torque RHS arm/1, D22/1, D12/1, D11/1
  Physical parameters/1 -> State torque parameters/3
  tau/1 -> State torque parameters/2
  x/1 -> State torque parameters/1

== system furuta_block_model_fixed_ppo_swingup/01 MIL - Controller and Plant/05 Furuta plant/RK4 Furuta plant/Substep 2/k1 ==
  x : Inport
  tau : Inport  Port=2
  Arm acceleration : Fcn  Expr=(u(3)*u(4)-u(2)*u(5))/(u(1)*u(3)-(u(2)*u(2)))
  Arm rate : Fcn  Expr=u(3)
  D11 : Fcn  Expr=u(6)+u(7)*(sin(u(2))*sin(u(2)))
  D12 : Fcn  Expr=u(9)*cos(u(2))
  D22 : Fcn  Expr=u(8)
  Mass matrix and RHS : Mux  Inputs=5
  Pend acceleration : Fcn  Expr=(u(1)*u(5)-u(2)*u(4))/(u(1)*u(3)-(u(2)*u(2)))
  Pend rate : Fcn  Expr=u(4)
  Physical parameters : Constant  Value=plantCoefficients
  State derivative : Mux
  State torque parameters : Mux  Inputs=3
  Torque RHS arm : Fcn  Expr=u(5)-2*u(7)*sin(u(2))*cos(u(2))*u(3)*u(4)+u(9)*sin(u(2))*(u(4)*u(4))-u(11)*u(3)-u(13)*sgn(u(3))
  Torque RHS pend : Fcn  Expr=u(7)*sin(u(2))*cos(u(2))*(u(3)*u(3))-u(12)*u(4)+u(10)*sin(u(2))
  xdot : Outport
  wires:
  State derivative/1 -> xdot/1
  Pend acceleration/1 -> State derivative/4
  Arm acceleration/1 -> State derivative/3
  Mass matrix and RHS/1 -> Pend acceleration/1, Arm acceleration/1
  Pend rate/1 -> State derivative/2
  Arm rate/1 -> State derivative/1
  Torque RHS pend/1 -> Mass matrix and RHS/5
  Torque RHS arm/1 -> Mass matrix and RHS/4
  D22/1 -> Mass matrix and RHS/3
  D12/1 -> Mass matrix and RHS/2
  D11/1 -> Mass matrix and RHS/1
  State torque parameters/1 -> Pend rate/1, Arm rate/1, Torque RHS pend/1, Torque RHS arm/1, D22/1, D12/1, D11/1
  Physical parameters/1 -> State torque parameters/3
  tau/1 -> State torque parameters/2
  x/1 -> State torque parameters/1

== system furuta_block_model_fixed_ppo_swingup/01 MIL - Controller and Plant/05 Furuta plant/RK4 Furuta plant/Substep 2/k2 ==
  x : Inport
  tau : Inport  Port=2
  Arm acceleration : Fcn  Expr=(u(3)*u(4)-u(2)*u(5))/(u(1)*u(3)-(u(2)*u(2)))
  Arm rate : Fcn  Expr=u(3)
  D11 : Fcn  Expr=u(6)+u(7)*(sin(u(2))*sin(u(2)))
  D12 : Fcn  Expr=u(9)*cos(u(2))
  D22 : Fcn  Expr=u(8)
  Mass matrix and RHS : Mux  Inputs=5
  Pend acceleration : Fcn  Expr=(u(1)*u(5)-u(2)*u(4))/(u(1)*u(3)-(u(2)*u(2)))
  Pend rate : Fcn  Expr=u(4)
  Physical parameters : Constant  Value=plantCoefficients
  State derivative : Mux
  State torque parameters : Mux  Inputs=3
  Torque RHS arm : Fcn  Expr=u(5)-2*u(7)*sin(u(2))*cos(u(2))*u(3)*u(4)+u(9)*sin(u(2))*(u(4)*u(4))-u(11)*u(3)-u(13)*sgn(u(3))
  Torque RHS pend : Fcn  Expr=u(7)*sin(u(2))*cos(u(2))*(u(3)*u(3))-u(12)*u(4)+u(10)*sin(u(2))
  xdot : Outport
  wires:
  x/1 -> State torque parameters/1
  tau/1 -> State torque parameters/2
  Physical parameters/1 -> State torque parameters/3
  State torque parameters/1 -> Arm rate/1, Pend rate/1, Torque RHS pend/1, Torque RHS arm/1, D22/1, D11/1, D12/1
  D11/1 -> Mass matrix and RHS/1
  D12/1 -> Mass matrix and RHS/2
  D22/1 -> Mass matrix and RHS/3
  Torque RHS arm/1 -> Mass matrix and RHS/4
  Torque RHS pend/1 -> Mass matrix and RHS/5
  Arm rate/1 -> State derivative/1
  Pend rate/1 -> State derivative/2
  Mass matrix and RHS/1 -> Arm acceleration/1, Pend acceleration/1
  Arm acceleration/1 -> State derivative/3
  Pend acceleration/1 -> State derivative/4
  State derivative/1 -> xdot/1

== system furuta_block_model_fixed_ppo_swingup/01 MIL - Controller and Plant/05 Furuta plant/RK4 Furuta plant/Substep 2/k3 ==
  x : Inport
  tau : Inport  Port=2
  Arm acceleration : Fcn  Expr=(u(3)*u(4)-u(2)*u(5))/(u(1)*u(3)-(u(2)*u(2)))
  Arm rate : Fcn  Expr=u(3)
  D11 : Fcn  Expr=u(6)+u(7)*(sin(u(2))*sin(u(2)))
  D12 : Fcn  Expr=u(9)*cos(u(2))
  D22 : Fcn  Expr=u(8)
  Mass matrix and RHS : Mux  Inputs=5
  Pend acceleration : Fcn  Expr=(u(1)*u(5)-u(2)*u(4))/(u(1)*u(3)-(u(2)*u(2)))
  Pend rate : Fcn  Expr=u(4)
  Physical parameters : Constant  Value=plantCoefficients
  State derivative : Mux
  State torque parameters : Mux  Inputs=3
  Torque RHS arm : Fcn  Expr=u(5)-2*u(7)*sin(u(2))*cos(u(2))*u(3)*u(4)+u(9)*sin(u(2))*(u(4)*u(4))-u(11)*u(3)-u(13)*sgn(u(3))
  Torque RHS pend : Fcn  Expr=u(7)*sin(u(2))*cos(u(2))*(u(3)*u(3))-u(12)*u(4)+u(10)*sin(u(2))
  xdot : Outport
  wires:
  x/1 -> State torque parameters/1
  tau/1 -> State torque parameters/2
  Physical parameters/1 -> State torque parameters/3
  State torque parameters/1 -> Arm rate/1, Pend rate/1, Torque RHS pend/1, Torque RHS arm/1, D22/1, D11/1, D12/1
  D11/1 -> Mass matrix and RHS/1
  D12/1 -> Mass matrix and RHS/2
  D22/1 -> Mass matrix and RHS/3
  Torque RHS arm/1 -> Mass matrix and RHS/4
  Torque RHS pend/1 -> Mass matrix and RHS/5
  Arm rate/1 -> State derivative/1
  Pend rate/1 -> State derivative/2
  Mass matrix and RHS/1 -> Arm acceleration/1, Pend acceleration/1
  Arm acceleration/1 -> State derivative/3
  Pend acceleration/1 -> State derivative/4
  State derivative/1 -> xdot/1

== system furuta_block_model_fixed_ppo_swingup/01 MIL - Controller and Plant/05 Furuta plant/RK4 Furuta plant/Substep 2/k4 ==
  x : Inport
  tau : Inport  Port=2
  Arm acceleration : Fcn  Expr=(u(3)*u(4)-u(2)*u(5))/(u(1)*u(3)-(u(2)*u(2)))
  Arm rate : Fcn  Expr=u(3)
  D11 : Fcn  Expr=u(6)+u(7)*(sin(u(2))*sin(u(2)))
  D12 : Fcn  Expr=u(9)*cos(u(2))
  D22 : Fcn  Expr=u(8)
  Mass matrix and RHS : Mux  Inputs=5
  Pend acceleration : Fcn  Expr=(u(1)*u(5)-u(2)*u(4))/(u(1)*u(3)-(u(2)*u(2)))
  Pend rate : Fcn  Expr=u(4)
  Physical parameters : Constant  Value=plantCoefficients
  State derivative : Mux
  State torque parameters : Mux  Inputs=3
  Torque RHS arm : Fcn  Expr=u(5)-2*u(7)*sin(u(2))*cos(u(2))*u(3)*u(4)+u(9)*sin(u(2))*(u(4)*u(4))-u(11)*u(3)-u(13)*sgn(u(3))
  Torque RHS pend : Fcn  Expr=u(7)*sin(u(2))*cos(u(2))*(u(3)*u(3))-u(12)*u(4)+u(10)*sin(u(2))
  xdot : Outport
  wires:
  x/1 -> State torque parameters/1
  tau/1 -> State torque parameters/2
  Physical parameters/1 -> State torque parameters/3
  State torque parameters/1 -> Arm rate/1, Pend rate/1, Torque RHS pend/1, Torque RHS arm/1, D22/1, D11/1, D12/1
  D11/1 -> Mass matrix and RHS/1
  D12/1 -> Mass matrix and RHS/2
  D22/1 -> Mass matrix and RHS/3
  Torque RHS arm/1 -> Mass matrix and RHS/4
  Torque RHS pend/1 -> Mass matrix and RHS/5
  Arm rate/1 -> State derivative/1
  Pend rate/1 -> State derivative/2
  Mass matrix and RHS/1 -> Arm acceleration/1, Pend acceleration/1
  Arm acceleration/1 -> State derivative/3
  Pend acceleration/1 -> State derivative/4
  State derivative/1 -> xdot/1

== system furuta_block_model_fixed_ppo_swingup/01 MIL - Controller and Plant/05 Furuta plant/RK4 Furuta plant/Substep 3/k1 ==
  x : Inport
  tau : Inport  Port=2
  Arm acceleration : Fcn  Expr=(u(3)*u(4)-u(2)*u(5))/(u(1)*u(3)-(u(2)*u(2)))
  Arm rate : Fcn  Expr=u(3)
  D11 : Fcn  Expr=u(6)+u(7)*(sin(u(2))*sin(u(2)))
  D12 : Fcn  Expr=u(9)*cos(u(2))
  D22 : Fcn  Expr=u(8)
  Mass matrix and RHS : Mux  Inputs=5
  Pend acceleration : Fcn  Expr=(u(1)*u(5)-u(2)*u(4))/(u(1)*u(3)-(u(2)*u(2)))
  Pend rate : Fcn  Expr=u(4)
  Physical parameters : Constant  Value=plantCoefficients
  State derivative : Mux
  State torque parameters : Mux  Inputs=3
  Torque RHS arm : Fcn  Expr=u(5)-2*u(7)*sin(u(2))*cos(u(2))*u(3)*u(4)+u(9)*sin(u(2))*(u(4)*u(4))-u(11)*u(3)-u(13)*sgn(u(3))
  Torque RHS pend : Fcn  Expr=u(7)*sin(u(2))*cos(u(2))*(u(3)*u(3))-u(12)*u(4)+u(10)*sin(u(2))
  xdot : Outport
  wires:
  State derivative/1 -> xdot/1
  Pend acceleration/1 -> State derivative/4
  Arm acceleration/1 -> State derivative/3
  Mass matrix and RHS/1 -> Pend acceleration/1, Arm acceleration/1
  Pend rate/1 -> State derivative/2
  Arm rate/1 -> State derivative/1
  Torque RHS pend/1 -> Mass matrix and RHS/5
  Torque RHS arm/1 -> Mass matrix and RHS/4
  D22/1 -> Mass matrix and RHS/3
  D12/1 -> Mass matrix and RHS/2
  D11/1 -> Mass matrix and RHS/1
  State torque parameters/1 -> Pend rate/1, Arm rate/1, Torque RHS pend/1, Torque RHS arm/1, D22/1, D12/1, D11/1
  Physical parameters/1 -> State torque parameters/3
  tau/1 -> State torque parameters/2
  x/1 -> State torque parameters/1

== system furuta_block_model_fixed_ppo_swingup/01 MIL - Controller and Plant/05 Furuta plant/RK4 Furuta plant/Substep 3/k2 ==
  x : Inport
  tau : Inport  Port=2
  Arm acceleration : Fcn  Expr=(u(3)*u(4)-u(2)*u(5))/(u(1)*u(3)-(u(2)*u(2)))
  Arm rate : Fcn  Expr=u(3)
  D11 : Fcn  Expr=u(6)+u(7)*(sin(u(2))*sin(u(2)))
  D12 : Fcn  Expr=u(9)*cos(u(2))
  D22 : Fcn  Expr=u(8)
  Mass matrix and RHS : Mux  Inputs=5
  Pend acceleration : Fcn  Expr=(u(1)*u(5)-u(2)*u(4))/(u(1)*u(3)-(u(2)*u(2)))
  Pend rate : Fcn  Expr=u(4)
  Physical parameters : Constant  Value=plantCoefficients
  State derivative : Mux
  State torque parameters : Mux  Inputs=3
  Torque RHS arm : Fcn  Expr=u(5)-2*u(7)*sin(u(2))*cos(u(2))*u(3)*u(4)+u(9)*sin(u(2))*(u(4)*u(4))-u(11)*u(3)-u(13)*sgn(u(3))
  Torque RHS pend : Fcn  Expr=u(7)*sin(u(2))*cos(u(2))*(u(3)*u(3))-u(12)*u(4)+u(10)*sin(u(2))
  xdot : Outport
  wires:
  x/1 -> State torque parameters/1
  tau/1 -> State torque parameters/2
  Physical parameters/1 -> State torque parameters/3
  State torque parameters/1 -> Arm rate/1, Pend rate/1, Torque RHS pend/1, Torque RHS arm/1, D22/1, D11/1, D12/1
  D11/1 -> Mass matrix and RHS/1
  D12/1 -> Mass matrix and RHS/2
  D22/1 -> Mass matrix and RHS/3
  Torque RHS arm/1 -> Mass matrix and RHS/4
  Torque RHS pend/1 -> Mass matrix and RHS/5
  Arm rate/1 -> State derivative/1
  Pend rate/1 -> State derivative/2
  Mass matrix and RHS/1 -> Arm acceleration/1, Pend acceleration/1
  Arm acceleration/1 -> State derivative/3
  Pend acceleration/1 -> State derivative/4
  State derivative/1 -> xdot/1

== system furuta_block_model_fixed_ppo_swingup/01 MIL - Controller and Plant/05 Furuta plant/RK4 Furuta plant/Substep 3/k3 ==
  x : Inport
  tau : Inport  Port=2
  Arm acceleration : Fcn  Expr=(u(3)*u(4)-u(2)*u(5))/(u(1)*u(3)-(u(2)*u(2)))
  Arm rate : Fcn  Expr=u(3)
  D11 : Fcn  Expr=u(6)+u(7)*(sin(u(2))*sin(u(2)))
  D12 : Fcn  Expr=u(9)*cos(u(2))
  D22 : Fcn  Expr=u(8)
  Mass matrix and RHS : Mux  Inputs=5
  Pend acceleration : Fcn  Expr=(u(1)*u(5)-u(2)*u(4))/(u(1)*u(3)-(u(2)*u(2)))
  Pend rate : Fcn  Expr=u(4)
  Physical parameters : Constant  Value=plantCoefficients
  State derivative : Mux
  State torque parameters : Mux  Inputs=3
  Torque RHS arm : Fcn  Expr=u(5)-2*u(7)*sin(u(2))*cos(u(2))*u(3)*u(4)+u(9)*sin(u(2))*(u(4)*u(4))-u(11)*u(3)-u(13)*sgn(u(3))
  Torque RHS pend : Fcn  Expr=u(7)*sin(u(2))*cos(u(2))*(u(3)*u(3))-u(12)*u(4)+u(10)*sin(u(2))
  xdot : Outport
  wires:
  x/1 -> State torque parameters/1
  tau/1 -> State torque parameters/2
  Physical parameters/1 -> State torque parameters/3
  State torque parameters/1 -> Arm rate/1, Pend rate/1, Torque RHS pend/1, Torque RHS arm/1, D22/1, D11/1, D12/1
  D11/1 -> Mass matrix and RHS/1
  D12/1 -> Mass matrix and RHS/2
  D22/1 -> Mass matrix and RHS/3
  Torque RHS arm/1 -> Mass matrix and RHS/4
  Torque RHS pend/1 -> Mass matrix and RHS/5
  Arm rate/1 -> State derivative/1
  Pend rate/1 -> State derivative/2
  Mass matrix and RHS/1 -> Arm acceleration/1, Pend acceleration/1
  Arm acceleration/1 -> State derivative/3
  Pend acceleration/1 -> State derivative/4
  State derivative/1 -> xdot/1

== system furuta_block_model_fixed_ppo_swingup/01 MIL - Controller and Plant/05 Furuta plant/RK4 Furuta plant/Substep 3/k4 ==
  x : Inport
  tau : Inport  Port=2
  Arm acceleration : Fcn  Expr=(u(3)*u(4)-u(2)*u(5))/(u(1)*u(3)-(u(2)*u(2)))
  Arm rate : Fcn  Expr=u(3)
  D11 : Fcn  Expr=u(6)+u(7)*(sin(u(2))*sin(u(2)))
  D12 : Fcn  Expr=u(9)*cos(u(2))
  D22 : Fcn  Expr=u(8)
  Mass matrix and RHS : Mux  Inputs=5
  Pend acceleration : Fcn  Expr=(u(1)*u(5)-u(2)*u(4))/(u(1)*u(3)-(u(2)*u(2)))
  Pend rate : Fcn  Expr=u(4)
  Physical parameters : Constant  Value=plantCoefficients
  State derivative : Mux
  State torque parameters : Mux  Inputs=3
  Torque RHS arm : Fcn  Expr=u(5)-2*u(7)*sin(u(2))*cos(u(2))*u(3)*u(4)+u(9)*sin(u(2))*(u(4)*u(4))-u(11)*u(3)-u(13)*sgn(u(3))
  Torque RHS pend : Fcn  Expr=u(7)*sin(u(2))*cos(u(2))*(u(3)*u(3))-u(12)*u(4)+u(10)*sin(u(2))
  xdot : Outport
  wires:
  x/1 -> State torque parameters/1
  tau/1 -> State torque parameters/2
  Physical parameters/1 -> State torque parameters/3
  State torque parameters/1 -> Arm rate/1, Pend rate/1, Torque RHS pend/1, Torque RHS arm/1, D22/1, D11/1, D12/1
  D11/1 -> Mass matrix and RHS/1
  D12/1 -> Mass matrix and RHS/2
  D22/1 -> Mass matrix and RHS/3
  Torque RHS arm/1 -> Mass matrix and RHS/4
  Torque RHS pend/1 -> Mass matrix and RHS/5
  Arm rate/1 -> State derivative/1
  Pend rate/1 -> State derivative/2
  Mass matrix and RHS/1 -> Arm acceleration/1, Pend acceleration/1
  Arm acceleration/1 -> State derivative/3
  Pend acceleration/1 -> State derivative/4
  State derivative/1 -> xdot/1

== system furuta_block_model_fixed_ppo_swingup/01 MIL - Controller and Plant/05 Furuta plant/RK4 Furuta plant/Substep 4/k1 ==
  x : Inport
  tau : Inport  Port=2
  Arm acceleration : Fcn  Expr=(u(3)*u(4)-u(2)*u(5))/(u(1)*u(3)-(u(2)*u(2)))
  Arm rate : Fcn  Expr=u(3)
  D11 : Fcn  Expr=u(6)+u(7)*(sin(u(2))*sin(u(2)))
  D12 : Fcn  Expr=u(9)*cos(u(2))
  D22 : Fcn  Expr=u(8)
  Mass matrix and RHS : Mux  Inputs=5
  Pend acceleration : Fcn  Expr=(u(1)*u(5)-u(2)*u(4))/(u(1)*u(3)-(u(2)*u(2)))
  Pend rate : Fcn  Expr=u(4)
  Physical parameters : Constant  Value=plantCoefficients
  State derivative : Mux
  State torque parameters : Mux  Inputs=3
  Torque RHS arm : Fcn  Expr=u(5)-2*u(7)*sin(u(2))*cos(u(2))*u(3)*u(4)+u(9)*sin(u(2))*(u(4)*u(4))-u(11)*u(3)-u(13)*sgn(u(3))
  Torque RHS pend : Fcn  Expr=u(7)*sin(u(2))*cos(u(2))*(u(3)*u(3))-u(12)*u(4)+u(10)*sin(u(2))
  xdot : Outport
  wires:
  State derivative/1 -> xdot/1
  Pend acceleration/1 -> State derivative/4
  Arm acceleration/1 -> State derivative/3
  Mass matrix and RHS/1 -> Pend acceleration/1, Arm acceleration/1
  Pend rate/1 -> State derivative/2
  Arm rate/1 -> State derivative/1
  Torque RHS pend/1 -> Mass matrix and RHS/5
  Torque RHS arm/1 -> Mass matrix and RHS/4
  D22/1 -> Mass matrix and RHS/3
  D12/1 -> Mass matrix and RHS/2
  D11/1 -> Mass matrix and RHS/1
  State torque parameters/1 -> Pend rate/1, Arm rate/1, Torque RHS pend/1, Torque RHS arm/1, D22/1, D12/1, D11/1
  Physical parameters/1 -> State torque parameters/3
  tau/1 -> State torque parameters/2
  x/1 -> State torque parameters/1

== system furuta_block_model_fixed_ppo_swingup/01 MIL - Controller and Plant/05 Furuta plant/RK4 Furuta plant/Substep 4/k2 ==
  x : Inport
  tau : Inport  Port=2
  Arm acceleration : Fcn  Expr=(u(3)*u(4)-u(2)*u(5))/(u(1)*u(3)-(u(2)*u(2)))
  Arm rate : Fcn  Expr=u(3)
  D11 : Fcn  Expr=u(6)+u(7)*(sin(u(2))*sin(u(2)))
  D12 : Fcn  Expr=u(9)*cos(u(2))
  D22 : Fcn  Expr=u(8)
  Mass matrix and RHS : Mux  Inputs=5
  Pend acceleration : Fcn  Expr=(u(1)*u(5)-u(2)*u(4))/(u(1)*u(3)-(u(2)*u(2)))
  Pend rate : Fcn  Expr=u(4)
  Physical parameters : Constant  Value=plantCoefficients
  State derivative : Mux
  State torque parameters : Mux  Inputs=3
  Torque RHS arm : Fcn  Expr=u(5)-2*u(7)*sin(u(2))*cos(u(2))*u(3)*u(4)+u(9)*sin(u(2))*(u(4)*u(4))-u(11)*u(3)-u(13)*sgn(u(3))
  Torque RHS pend : Fcn  Expr=u(7)*sin(u(2))*cos(u(2))*(u(3)*u(3))-u(12)*u(4)+u(10)*sin(u(2))
  xdot : Outport
  wires:
  x/1 -> State torque parameters/1
  tau/1 -> State torque parameters/2
  Physical parameters/1 -> State torque parameters/3
  State torque parameters/1 -> Arm rate/1, Pend rate/1, Torque RHS pend/1, Torque RHS arm/1, D22/1, D11/1, D12/1
  D11/1 -> Mass matrix and RHS/1
  D12/1 -> Mass matrix and RHS/2
  D22/1 -> Mass matrix and RHS/3
  Torque RHS arm/1 -> Mass matrix and RHS/4
  Torque RHS pend/1 -> Mass matrix and RHS/5
  Arm rate/1 -> State derivative/1
  Pend rate/1 -> State derivative/2
  Mass matrix and RHS/1 -> Arm acceleration/1, Pend acceleration/1
  Arm acceleration/1 -> State derivative/3
  Pend acceleration/1 -> State derivative/4
  State derivative/1 -> xdot/1
